simulink model "attitude_loop"  (R2026b)
settings: Solver=VariableStepAuto
undefined symbols (not defined in the file): p
settings Model: Creator=lorenzomonti  LastModifiedBy=lorenzomonti

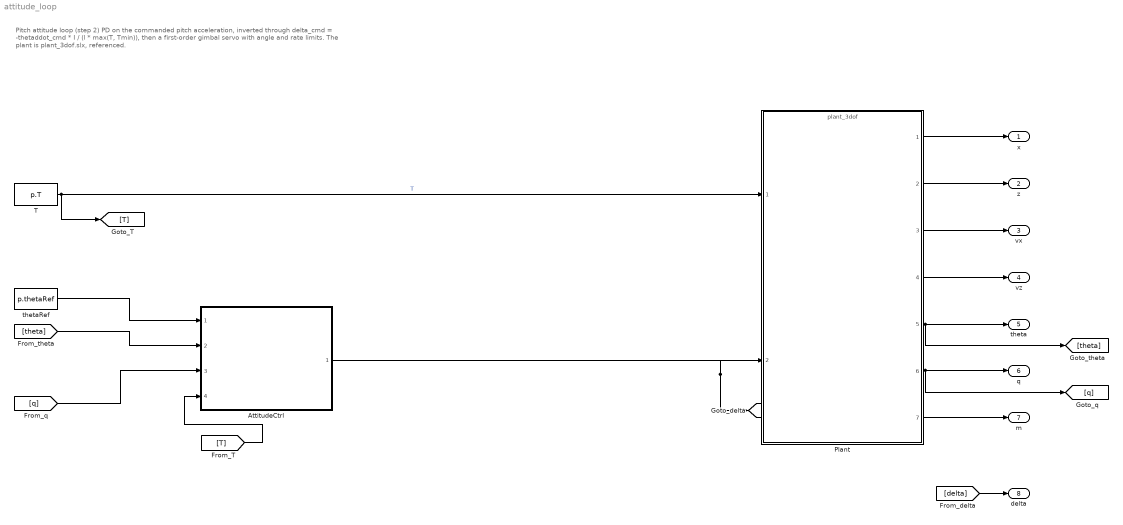
== system attitude_loop ==
  note: Pitch attitude loop (step 2)
      | PD on the commanded pitch acceleration, inverted through delta_cmd = -thetaddot_cmd * I / (l * max(T, Tmin)),
      | then a first-order gimbal servo with angle and rate limits. The plant is plant_3dof.slx, referenced.
  AttitudeCtrl : Subsystem  ReferencedSubsystem=attitude_ctrl
  Plant : ModelReference  ModelNameDialog=plant_3dof  SimulationMode=Normal  ModelReferenceVersion=1.16
  T : Constant  Value=p.T
  thetaRef : Constant  Value=p.thetaRef
  x : Outport
  z : Outport  Port=2
  vx : Outport  Port=3
  vz : Outport  Port=4
  theta : Outport  Port=5
  q : Outport  Port=6
  m : Outport  Port=7
  delta : Outport  Port=8
  wires:
  T/1 -> Plant/1, [T]  "T"
  [delta] -> delta/1
  Plant/1 -> x/1
  Plant/2 -> z/1
  Plant/3 -> vx/1
  Plant/4 -> vz/1
  Plant/5 -> theta/1, [theta]
  Plant/6 -> q/1, [q]
  Plant/7 -> m/1
  AttitudeCtrl/1 -> Plant/2, [delta]
  thetaRef/1 -> AttitudeCtrl/1
  [theta] -> AttitudeCtrl/2
  [q] -> AttitudeCtrl/3
  [T] -> AttitudeCtrl/4
